simulink model "Robust_LQR"  (R2024a)
settings: Solver=VariableStepAuto  StartTime=0.0  StopTime=10  FixedStep=0.01  RelTol=1e-3
libraries: instrumentseriallib x3, simulink x1
settings Model: Creator=S I N O  LastModifiedBy=S I N O

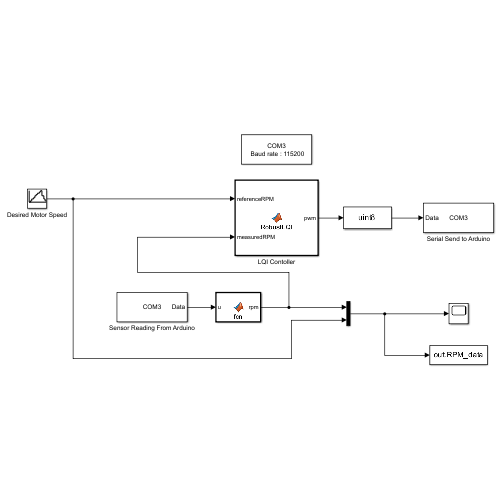
[thumbnail: Simulink's stored preview of the top-level diagram]
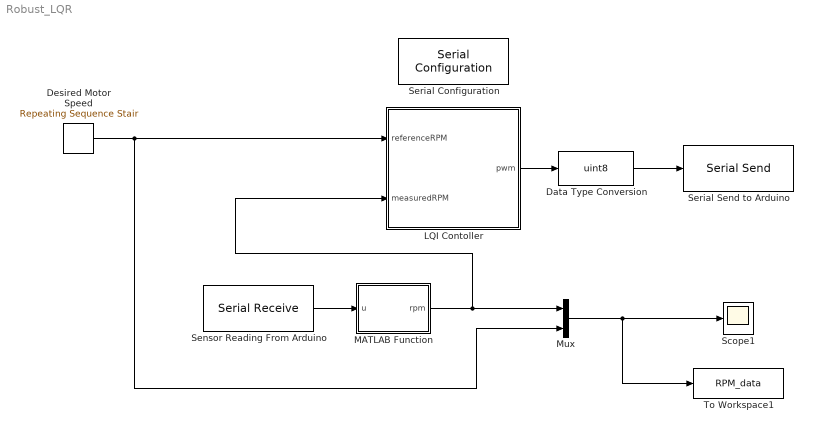
== system Robust_LQR ==
  Data Type Conversion : DataTypeConversion  OutDataTypeStr=uint8  SaturateOnIntegerOverflow=off  RndMeth=Floor
  Desired Motor Speed : simulink/Sources/Repeating Sequence Stair  OutValues=[0 500 1000 1500 2000 2500 3000 3500 4000 2000 1000 500].'  tsamp=0.8  OutMin=[]  OutMax=[]  OutDataTypeStr=double  OutputDataTypeScalingMode=double  OutDataType=fixdt(0,8)  ConRadixGroup=Best Precision: Vector-wise  OutScaling=2^-12
  LQI Contoller : MATLAB Function  TreatAsAtomicUnit=on
  MATLAB Function : MATLAB Function  TreatAsAtomicUnit=on
  Mux : Mux  Inputs=2
  Scope1 : Scope
  Sensor Reading From Arduino : instrumentseriallib/Serial Receive  PortSel=COM3  Port=COM3  ComPort=COM3  DataType=uint8  SaveDataType=uint8  ToggleHeader=off  Header=[]  ToggleDataSize=on  DataSize=2  ToggleTerminator=off  Terminator=<none>  CustomTerminator=[]  InputFormat=Column major  EnableBlockingMode=on  ActionDataUnavailable=Output last received value  ActionWhenDataUnavailable=Output last received value  CustomValue=0  SampleTime=0.01  SimulateUsing=Interpreted execution  BlockInModel=on  aMode=1
  Serial Configuration : instrumentseriallib/Serial Configuration  Priority=-200000  PortSel=COM3  Port=COM3  ComPort=COM3  BaudRate=115200  DataBits=8  Parity=none  StopBits=1  ByteOrder=little-endian  FlowControl=none  Timeout=1  SimulateUsing=Interpreted execution  BlockInModel=on  aMode=1
  Serial Send to Arduino : instrumentseriallib/Serial Send  PortSel=COM3  Port=COM3  ComPort=COM3  Header=[]  Terminator=<none>  CustomTerminator=[]  EnableBlockingMode=on  SimulateUsing=Interpreted execution  BlockInModel=on  aMode=1
  To Workspace1 : ToWorkspace  VariableName=RPM_data  SaveFormat=Timeseries  SampleTime=-1
  wires:
  Sensor Reading From Arduino/1 -> MATLAB Function/1(u)
  MATLAB Function/1(rpm) -> Mux/1, LQI Contoller/2(measuredRPM)
  Desired Motor Speed/1 -> LQI Contoller/1(referenceRPM), Mux/2
  LQI Contoller/1(pwm) -> Data Type Conversion/1
  Data Type Conversion/1 -> Serial Send to Arduino/1
  Mux/1 -> To Workspace1/1, Scope1/1

== matlab function Robust_LQR/MATLAB Function ==
  data: u input; rpm output
function rpm = fcn(u)

rpm = double(u(1))*256 + double(u(2));

end

== matlab function Robust_LQR/LQI Contoller ==
  data: referenceRPM input; pwm output; measuredRPM input
function pwm = RobustLQI(referenceRPM, measuredRPM)

    persistent integralError PWMmap RPMmap RPMu PWMu

    if isempty(integralError)
        integralError = 0;

scale = [0.1 0.1 0.1 0.1 0.1 0.1 0.1 0.1 0.1 0.1 ...
         0.1 0.1 0.1 0.1 0.1 0.1 0.1 0.1 0.1 0.1 ...
         0.40 0.42 0.45 0.45 0.45 0.45 0.45];

PWMmap = [0 10 20 30 40 50 60 70 80 90 ...
          100 110 120 130 140 150 160 170 180 190 ...
          200 210 220 230 240 250 255] .* scale;

        RPMmap = [0 0 0 20 200 440 720 980 1210 1410 ...
                  1600 1760 1910 2130 2430 2720 3010 3250 3430 3480 ...
                  3560 3680 3750 3800 3900 3990 4020];

        [RPMu, idx] = unique(RPMmap);
        PWMu = PWMmap(idx);
    end

    Ts = 0.01;
    Kx =  0.0012146284;
    Ki = -0.3474520864;

    error = referenceRPM - measuredRPM;

    % --- Candidate integral update ---
    integralCandidate = integralError + Ts * error;

    % --- Feedback law using the CANDIDATE integral ---
    u_fb = -Kx * measuredRPM - Ki * integralCandidate;

    % --- Feedforward ---
    ff = interp1(RPMu, PWMu, referenceRPM, 'linear', 'extrap');
    ff = min(max(ff, 0), 255);

    % --- Unconstrained (pre-saturation) command ---
    u = ff + u_fb;

    % --- Saturation delta ---
    u_sat    = min(max(u, 0), 255);
    deltaPWM = u_sat - u;   % >0 means we clipped upward, <0 means clipped downward

    % --- Conditional integration anti-windup ---
    if (u > 0 && u < 255) || ...
       (u >= 255 && deltaPWM < 0) || ...
       (u <= 0 && deltaPWM > 0)
        integralError = integralCandidate;
    end

    pwm = uint8(round(u_sat));
end
